simulink model "sensor_real_temp_LU"  (R2026b)
settings: Solver=VariableStepAuto
values from neighbouring files (symbols this model uses):
  init_Ts = 20    [coeficientes.m]
  tau_RTD = 20    [coeficientes.m]
settings Model: Creator=lamun  LastModifiedBy=lamun

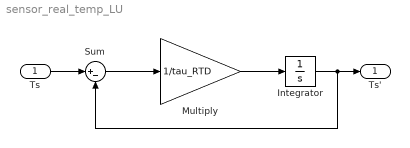
== system sensor_real_temp_LU ==
  Ts : Inport
  Integrator : Integrator  InitialCondition=init_Ts
  Multiply : Gain  Gain=1/tau_RTD
  Sum : Sum  Inputs=|+-
  Ts' : Outport
  wires:
  Multiply/1 -> Integrator/1
  Integrator/1 -> Sum/2, Ts'/1
  Sum/1 -> Multiply/1
  Ts/1 -> Sum/1
